simulink model "Dll_Control_AFO_V8_5_R2019b"  (R2019b)
settings: Solver=ode2  StartTime=0.0  StopTime=10  FixedStep=Ts  RelTol=1e-3
InitFcn:
  | modelDir=fileparts(get_param(bdroot,'FileName'));addpath(modelDir);rootDir=fileparts(modelDir);if isfolder(rootDir),addpath(rootDir);end;fmuDir=fullfile(rootDir,'fmu');if isfolder(fmuDir),addpath(fmuDir);end;if evalin('base','exist(''Wf0'',''var'')'),assignin('base','Wfb',evalin('base','Wf0'));end;
values from neighbouring files (symbols this model uses):
  A80 = 0.10573    [RunCtrlSysModelSHT.m]
  b11 = B(1,1)*1    [RunCtrlSysModelSHT.m]
  b21 = B(2,1)*1    [RunCtrlSysModelSHT.m]
  d31 = D(3,1)    [RunCtrlSysModelSHT.m]
  d41 = D(4,1)    [RunCtrlSysModelSHT.m]
  ExternalSecondaryAirEnabled = 0    [RunCtrlSysModelSHT.m]
  InitAir = zeros(50,1)    [RunCtrlSysModelSHT.m]
  Mkg0 = 0    [RunCtrlSysModelSHT.m]
  MkpDirectCommand = Mkp0    (= 999.278795578)    [RunCtrlSysModelSHT.m]
  MkpMax = 1200    [RunCtrlSysModelSHT.m]
  Ng0 = 38000    [RunCtrlSysModelSHT.m]
  NgMax = Ng0*1.05    (= 39900)    [RunCtrlSysModelSHT.m]
  Np0 = 20800    [RunCtrlSysModelSHT.m]
  NpDem = Np0    (= 20800)    [RunCtrlSysModelSHT.m]
  omega_u = 20    [RunCtrlSysModelSHT.m]
  power0 = 2176600    [RunCtrlSysModelSHT.m]
  RotorLoadCfg = struct(      'designNpRpm', Np0,      'designPowerW', power0,      'thetaZeroDeg', 0,      'thetaDesignDeg', 12,      'profileTorqueFraction', 0.15,      'thetaValidRangeDeg', [6, 14])    [RunCtrlSysModelSHT.m]
  RotorLoadInputMode = 'legacyPower'    [RunCtrlSysModelSHT.m]
  T45Max = 1400    [RunCtrlSysModelSHT.m]
  ThetaCommandDeg = RotorLoadCfg.thetaDesignDeg    [RunCtrlSysModelSHT.m]
  Ts = 0.025    [RunCtrlSysModelSHT.m]
  Wf0 = 0.151914044493225    (= 0.151914044493)    [RunCtrlSysModelSHT.m]
  WfMax = Wf0*2    (= 0.303828088986)    [RunCtrlSysModelSHT.m]
  WfMin = Wf0*0.01    (= 0.00151914044493)    [RunCtrlSysModelSHT.m]
  WfRateLim = 1.5    [RunCtrlSysModelSHT.m]
undefined symbols (not defined in the file or in its folder): sigbuilder_block, Wfb
libraries: simulink x10
(part 3 of 4)

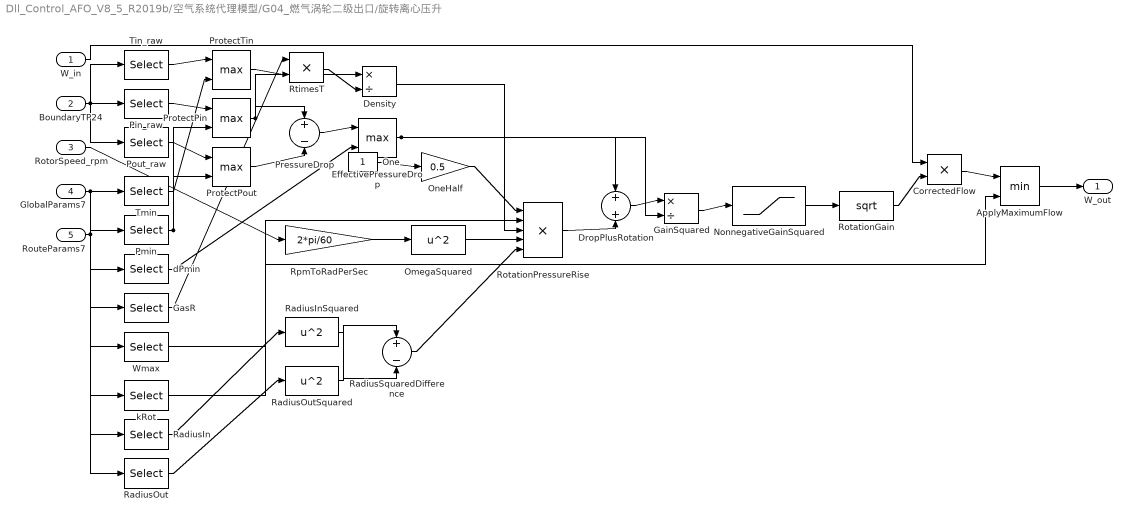
== system Dll_Control_AFO_V8_5_R2019b/空气系统代理模型/G04_燃气涡轮二级出口/旋转离心压升 ==
  W_in : Inport  PortDimensions=1
  BoundaryTP24 : Inport  Port=2  PortDimensions=24
  RotorSpeed_rpm : Inport  Port=3  PortDimensions=1
  GlobalParams7 : Inport  Port=4  PortDimensions=7
  RouteParams7 : Inport  Port=5  PortDimensions=7
  ApplyMaximumFlow : MinMax  Inputs=2
  CorrectedFlow : Product  Inputs=**
  Density : Product  Inputs=*/
  DropPlusRotation : Sum
  EffectivePressureDrop : MinMax  Function=max  Inputs=2
  GainSquared : Product  Inputs=*/
  GasR : Selector  InputPortWidth=7  IndexOptions=Index vector (dialog)  Indices=5  OutputSizes=1
  NonnegativeGainSquared : Saturate  UpperLimit=16  LowerLimit=0
  OmegaSquared : Math  Operator=square  SignedPower=off  SaturateOnIntegerOverflow=on
  One : Constant
  OneHalf : Gain  Gain=0.5
  Pin_raw : Selector  InputPortWidth=24  IndexOptions=Index vector (dialog)  Indices=2*UpstreamBoundary  OutputSizes=1
  Pmin : Selector  InputPortWidth=7  IndexOptions=Index vector (dialog)  Indices=2  OutputSizes=1
  Pout_raw : Selector  InputPortWidth=24  IndexOptions=Index vector (dialog)  Indices=2*DownstreamBoundary  OutputSizes=1
  PressureDrop : Sum  Inputs=+-
  ProtectPin : MinMax  Function=max  Inputs=2
  ProtectPout : MinMax  Function=max  Inputs=2
  ProtectTin : MinMax  Function=max  Inputs=2
  RadiusIn : Selector  InputPortWidth=7  IndexOptions=Index vector (dialog)  Indices=3  OutputSizes=1
  RadiusInSquared : Math  Operator=square  SignedPower=off  SaturateOnIntegerOverflow=on
  RadiusOut : Selector  InputPortWidth=7  IndexOptions=Index vector (dialog)  Indices=4  OutputSizes=1
  RadiusOutSquared : Math  Operator=square  SignedPower=off  SaturateOnIntegerOverflow=on
  RadiusSquaredDifference : Sum  Inputs=+-
  RotationGain : Math  Operator=sqrt  SignedPower=off  SaturateOnIntegerOverflow=on
  RotationPressureRise : Product  Inputs=*****
  RpmToRadPerSec : Gain  Gain=2*pi/60
  RtimesT : Product  Inputs=**
  Tin_raw : Selector  InputPortWidth=24  IndexOptions=Index vector (dialog)  Indices=2*UpstreamBoundary-1  OutputSizes=1
  Tmin : Selector  InputPortWidth=7  IndexOptions=Index vector (dialog)  Indices=1  OutputSizes=1
  Wmax : Selector  InputPortWidth=7  IndexOptions=Index vector (dialog)  Indices=6  OutputSizes=1
  dPmin : Selector  InputPortWidth=7  IndexOptions=Index vector (dialog)  Indices=3  OutputSizes=1
  kRot : Selector  InputPortWidth=7  IndexOptions=Index vector (dialog)  Indices=2  OutputSizes=1
  W_out : Outport
  wires:
  ApplyMaximumFlow/1 -> W_out/1
  Wmax/1 -> ApplyMaximumFlow/2
  CorrectedFlow/1 -> ApplyMaximumFlow/1
  RotationGain/1 -> CorrectedFlow/2
  W_in/1 -> CorrectedFlow/1
  NonnegativeGainSquared/1 -> RotationGain/1
  GainSquared/1 -> NonnegativeGainSquared/1
  DropPlusRotation/1 -> GainSquared/1
  RotationPressureRise/1 -> DropPlusRotation/2
  EffectivePressureDrop/1 -> GainSquared/2, DropPlusRotation/1
  dPmin/1 -> EffectivePressureDrop/2
  PressureDrop/1 -> EffectivePressureDrop/1
  ProtectPout/1 -> PressureDrop/2
  RadiusSquaredDifference/1 -> RotationPressureRise/5
  OmegaSquared/1 -> RotationPressureRise/4
  Density/1 -> RotationPressureRise/3
  kRot/1 -> RotationPressureRise/2
  OneHalf/1 -> RotationPressureRise/1
  One/1 -> OneHalf/1
  RadiusInSquared/1 -> RadiusSquaredDifference/2
  RadiusOutSquared/1 -> RadiusSquaredDifference/1
  RadiusOut/1 -> RadiusOutSquared/1
  RadiusIn/1 -> RadiusInSquared/1
  RpmToRadPerSec/1 -> OmegaSquared/1
  RotorSpeed_rpm/1 -> RpmToRadPerSec/1
  RtimesT/1 -> Density/2
  ProtectPin/1 -> PressureDrop/1, Density/1
  ProtectTin/1 -> RtimesT/2
  GasR/1 -> RtimesT/1
  Pout_raw/1 -> ProtectPout/1
  Pmin/1 -> ProtectPout/2, ProtectPin/2
  Pin_raw/1 -> ProtectPin/1
  Tmin/1 -> ProtectTin/2
  Tin_raw/1 -> ProtectTin/1
  RouteParams7/1 -> RadiusOut/1, RadiusIn/1, kRot/1
  GlobalParams7/1 -> Wmax/1, GasR/1, dPmin/1, Pmin/1, Tmin/1
  BoundaryTP24/1 -> Pout_raw/1, Pin_raw/1, Tin_raw/1

== system Dll_Control_AFO_V8_5_R2019b/空气系统代理模型/G04_燃气涡轮二级出口/流路可调参数 ==
  Mux_RouteParams7 : Mux  Inputs=7
  kRot : Constant  Value=0.5
  内半径_m : Constant  Value=0.074499999999999997
  初值流量_kgps : Constant  Value=0.099328741948656193
  外半径_m : Constant  Value=0.078
  时间常数_s : Constant  Value=0
  等效面积缩放 : Constant  Value=0.9867972125855029
  篦齿修正系数 : Constant
  RouteParams7 : Outport
  wires:
  等效面积缩放/1 -> Mux_RouteParams7/1
  kRot/1 -> Mux_RouteParams7/2
  内半径_m/1 -> Mux_RouteParams7/3
  外半径_m/1 -> Mux_RouteParams7/4
  时间常数_s/1 -> Mux_RouteParams7/5
  初值流量_kgps/1 -> Mux_RouteParams7/6
  篦齿修正系数/1 -> Mux_RouteParams7/7
  Mux_RouteParams7/1 -> RouteParams7/1

== system Dll_Control_AFO_V8_5_R2019b/空气系统代理模型/G04_燃气涡轮二级出口/辨识等效面积 ==
  BoundaryTP24 : Inport  PortDimensions=24
  IdentifiedAreaLaw : MATLAB Function  TreatAsAtomicUnit=on
  EffectiveArea_m2 : Outport
  wires:
  BoundaryTP24/1 -> IdentifiedAreaLaw/1(boundaryTP24)
  IdentifiedAreaLaw/1(area) -> EffectiveArea_m2/1

== system Dll_Control_AFO_V8_5_R2019b/空气系统代理模型/G05_动力涡轮一级叶根进口/可压缩节流孔口 ==
  BoundaryTP24 : Inport  PortDimensions=24
  EffectiveArea_m2 : Inport  Port=2  PortDimensions=1
  GlobalParams7 : Inport  Port=3  PortDimensions=7
  ApplyMaximumFlow : MinMax  Inputs=2
  BoundRatio : Saturate  UpperLimit=1  LowerLimit=1e-6
  CriticalEnabled : Selector  InputPortWidth=7  IndexOptions=Index vector (dialog)  Indices=7  OutputSizes=1
  CriticalRatio : Fcn  Expr=(2/(u+1))^(u/(u-1))
  EnableForwardFlow : Switch  Criteria=u2 ~= 0
  ForwardFlow : RelationalOperator  Operator=>  OutDataTypeStr=boolean  RndMeth=Simplest
  Gamma : Selector  InputPortWidth=7  IndexOptions=Index vector (dialog)  Indices=4  OutputSizes=1
  GasR : Selector  InputPortWidth=7  IndexOptions=Index vector (dialog)  Indices=5  OutputSizes=1
  IsChoked : RelationalOperator  Operator=<=  OutDataTypeStr=boolean  RndMeth=Simplest
  MassFlowRaw : Product  Inputs=***/
  MuxGammaRatio : Mux  Inputs=2
  PhiChoked : Fcn  Expr=sqrt(u)*(2/(u+1))^((u+1)/(2*(u-1)))
  PhiSubcritical : Fcn  Expr=sqrt(2*u(1)/(u(1)-1)*(u(2)^(2/u(1))-u(2)^((u(1)+1)/u(1))))
  Pin_raw : Selector  InputPortWidth=24  IndexOptions=Index vector (dialog)  Indices=2*UpstreamBoundary  OutputSizes=1
  Pmin : Selector  InputPortWidth=7  IndexOptions=Index vector (dialog)  Indices=2  OutputSizes=1
  PoutPlusMinimumDrop : Sum
  Pout_raw : Selector  InputPortWidth=24  IndexOptions=Index vector (dialog)  Indices=2*DownstreamBoundary  OutputSizes=1
  PressureRatio : Product  Inputs=*/
  ProtectPin : MinMax  Function=max  Inputs=2
  ProtectPout : MinMax  Function=max  Inputs=2
  ProtectTin : MinMax  Function=max  Inputs=2
  RT : Product  Inputs=**
  SelectPhi : Switch  Criteria=u2 ~= 0
  SqrtRT : Math  Operator=sqrt  SignedPower=off  SaturateOnIntegerOverflow=on
  Tin_raw : Selector  InputPortWidth=24  IndexOptions=Index vector (dialog)  Indices=2*UpstreamBoundary-1  OutputSizes=1
  Tmin : Selector  InputPortWidth=7  IndexOptions=Index vector (dialog)  Indices=1  OutputSizes=1
  UseChokedBranch : Logic  AllPortsSameDT=off  OutDataTypeStr=boolean
  Wmax : Selector  InputPortWidth=7  IndexOptions=Index vector (dialog)  Indices=6  OutputSizes=1
  ZeroFlow : Constant  Value=0
  dPmin : Selector  InputPortWidth=7  IndexOptions=Index vector (dialog)  Indices=3  OutputSizes=1
  W_kgps : Outport
  wires:
  ApplyMaximumFlow/1 -> W_kgps/1
  Wmax/1 -> ApplyMaximumFlow/2
  EnableForwardFlow/1 -> ApplyMaximumFlow/1
  ZeroFlow/1 -> EnableForwardFlow/3
  ForwardFlow/1 -> EnableForwardFlow/2
  MassFlowRaw/1 -> EnableForwardFlow/1
  SqrtRT/1 -> MassFlowRaw/4
  EffectiveArea_m2/1 -> MassFlowRaw/3
  SelectPhi/1 -> MassFlowRaw/2
  RT/1 -> SqrtRT/1
  ProtectTin/1 -> RT/2
  GasR/1 -> RT/1
  PhiSubcritical/1 -> SelectPhi/3
  UseChokedBranch/1 -> SelectPhi/2
  PhiChoked/1 -> SelectPhi/1
  CriticalEnabled/1 -> UseChokedBranch/2
  IsChoked/1 -> UseChokedBranch/1
  CriticalRatio/1 -> IsChoked/2
  MuxGammaRatio/1 -> PhiSubcritical/1
  BoundRatio/1 -> IsChoked/1, MuxGammaRatio/2
  Gamma/1 -> MuxGammaRatio/1, PhiChoked/1, CriticalRatio/1
  PressureRatio/1 -> BoundRatio/1
  PoutPlusMinimumDrop/1 -> ForwardFlow/2
  ProtectPin/1 -> MassFlowRaw/1, PressureRatio/2, ForwardFlow/1
  dPmin/1 -> PoutPlusMinimumDrop/2
  ProtectPout/1 -> PressureRatio/1, PoutPlusMinimumDrop/1
  Pout_raw/1 -> ProtectPout/1
  Pmin/1 -> ProtectPout/2, ProtectPin/2
  Pin_raw/1 -> ProtectPin/1
  Tmin/1 -> ProtectTin/2
  Tin_raw/1 -> ProtectTin/1
  GlobalParams7/1 -> CriticalEnabled/1, Wmax/1, GasR/1, Gamma/1, dPmin/1, Pmin/1, Tmin/1
  BoundaryTP24/1 -> Pout_raw/1, Pin_raw/1, Tin_raw/1

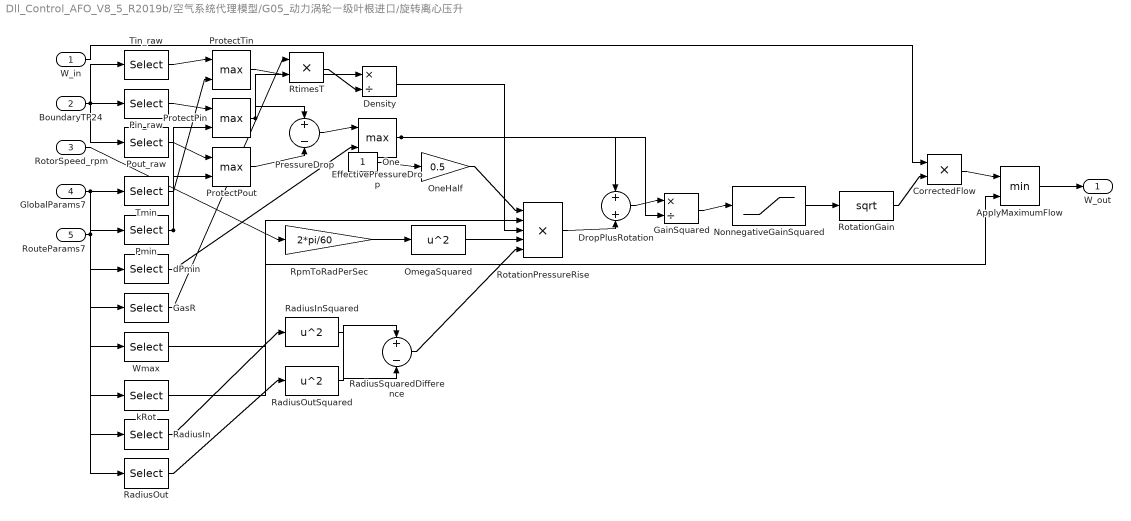
== system Dll_Control_AFO_V8_5_R2019b/空气系统代理模型/G05_动力涡轮一级叶根进口/旋转离心压升 ==
  W_in : Inport  PortDimensions=1
  BoundaryTP24 : Inport  Port=2  PortDimensions=24
  RotorSpeed_rpm : Inport  Port=3  PortDimensions=1
  GlobalParams7 : Inport  Port=4  PortDimensions=7
  RouteParams7 : Inport  Port=5  PortDimensions=7
  ApplyMaximumFlow : MinMax  Inputs=2
  CorrectedFlow : Product  Inputs=**
  Density : Product  Inputs=*/
  DropPlusRotation : Sum
  EffectivePressureDrop : MinMax  Function=max  Inputs=2
  GainSquared : Product  Inputs=*/
  GasR : Selector  InputPortWidth=7  IndexOptions=Index vector (dialog)  Indices=5  OutputSizes=1
  NonnegativeGainSquared : Saturate  UpperLimit=16  LowerLimit=0
  OmegaSquared : Math  Operator=square  SignedPower=off  SaturateOnIntegerOverflow=on
  One : Constant
  OneHalf : Gain  Gain=0.5
  Pin_raw : Selector  InputPortWidth=24  IndexOptions=Index vector (dialog)  Indices=2*UpstreamBoundary  OutputSizes=1
  Pmin : Selector  InputPortWidth=7  IndexOptions=Index vector (dialog)  Indices=2  OutputSizes=1
  Pout_raw : Selector  InputPortWidth=24  IndexOptions=Index vector (dialog)  Indices=2*DownstreamBoundary  OutputSizes=1
  PressureDrop : Sum  Inputs=+-
  ProtectPin : MinMax  Function=max  Inputs=2
  ProtectPout : MinMax  Function=max  Inputs=2
  ProtectTin : MinMax  Function=max  Inputs=2
  RadiusIn : Selector  InputPortWidth=7  IndexOptions=Index vector (dialog)  Indices=3  OutputSizes=1
  RadiusInSquared : Math  Operator=square  SignedPower=off  SaturateOnIntegerOverflow=on
  RadiusOut : Selector  InputPortWidth=7  IndexOptions=Index vector (dialog)  Indices=4  OutputSizes=1
  RadiusOutSquared : Math  Operator=square  SignedPower=off  SaturateOnIntegerOverflow=on
  RadiusSquaredDifference : Sum  Inputs=+-
  RotationGain : Math  Operator=sqrt  SignedPower=off  SaturateOnIntegerOverflow=on
  RotationPressureRise : Product  Inputs=*****
  RpmToRadPerSec : Gain  Gain=2*pi/60
  RtimesT : Product  Inputs=**
  Tin_raw : Selector  InputPortWidth=24  IndexOptions=Index vector (dialog)  Indices=2*UpstreamBoundary-1  OutputSizes=1
  Tmin : Selector  InputPortWidth=7  IndexOptions=Index vector (dialog)  Indices=1  OutputSizes=1
  Wmax : Selector  InputPortWidth=7  IndexOptions=Index vector (dialog)  Indices=6  OutputSizes=1
  dPmin : Selector  InputPortWidth=7  IndexOptions=Index vector (dialog)  Indices=3  OutputSizes=1
  kRot : Selector  InputPortWidth=7  IndexOptions=Index vector (dialog)  Indices=2  OutputSizes=1
  W_out : Outport
  wires:
  ApplyMaximumFlow/1 -> W_out/1
  Wmax/1 -> ApplyMaximumFlow/2
  CorrectedFlow/1 -> ApplyMaximumFlow/1
  RotationGain/1 -> CorrectedFlow/2
  W_in/1 -> CorrectedFlow/1
  NonnegativeGainSquared/1 -> RotationGain/1
  GainSquared/1 -> NonnegativeGainSquared/1
  DropPlusRotation/1 -> GainSquared/1
  RotationPressureRise/1 -> DropPlusRotation/2
  EffectivePressureDrop/1 -> GainSquared/2, DropPlusRotation/1
  dPmin/1 -> EffectivePressureDrop/2
  PressureDrop/1 -> EffectivePressureDrop/1
  ProtectPout/1 -> PressureDrop/2
  RadiusSquaredDifference/1 -> RotationPressureRise/5
  OmegaSquared/1 -> RotationPressureRise/4
  Density/1 -> RotationPressureRise/3
  kRot/1 -> RotationPressureRise/2
  OneHalf/1 -> RotationPressureRise/1
  One/1 -> OneHalf/1
  RadiusInSquared/1 -> RadiusSquaredDifference/2
  RadiusOutSquared/1 -> RadiusSquaredDifference/1
  RadiusOut/1 -> RadiusOutSquared/1
  RadiusIn/1 -> RadiusInSquared/1
  RpmToRadPerSec/1 -> OmegaSquared/1
  RotorSpeed_rpm/1 -> RpmToRadPerSec/1
  RtimesT/1 -> Density/2
  ProtectPin/1 -> PressureDrop/1, Density/1
  ProtectTin/1 -> RtimesT/2
  GasR/1 -> RtimesT/1
  Pout_raw/1 -> ProtectPout/1
  Pmin/1 -> ProtectPout/2, ProtectPin/2
  Pin_raw/1 -> ProtectPin/1
  Tmin/1 -> ProtectTin/2
  Tin_raw/1 -> ProtectTin/1
  RouteParams7/1 -> RadiusOut/1, RadiusIn/1, kRot/1
  GlobalParams7/1 -> Wmax/1, GasR/1, dPmin/1, Pmin/1, Tmin/1
  BoundaryTP24/1 -> Pout_raw/1, Pin_raw/1, Tin_raw/1

== system Dll_Control_AFO_V8_5_R2019b/空气系统代理模型/G05_动力涡轮一级叶根进口/流路可调参数 ==
  Mux_RouteParams7 : Mux  Inputs=7
  kRot : Constant  Value=0.5
  内半径_m : Constant  Value=0.053999999999999999
  初值流量_kgps : Constant  Value=0.038254988453198698
  外半径_m : Constant  Value=0.059499999999999997
  时间常数_s : Constant  Value=0
  等效面积缩放 : Constant  Value=0.989491921844591
  篦齿修正系数 : Constant
  RouteParams7 : Outport
  wires:
  等效面积缩放/1 -> Mux_RouteParams7/1
  kRot/1 -> Mux_RouteParams7/2
  内半径_m/1 -> Mux_RouteParams7/3
  外半径_m/1 -> Mux_RouteParams7/4
  时间常数_s/1 -> Mux_RouteParams7/5
  初值流量_kgps/1 -> Mux_RouteParams7/6
  篦齿修正系数/1 -> Mux_RouteParams7/7
  Mux_RouteParams7/1 -> RouteParams7/1

== system Dll_Control_AFO_V8_5_R2019b/空气系统代理模型/G05_动力涡轮一级叶根进口/盘腔热动态 ==
  W_in : Inport  PortDimensions=1
  RouteParams7 : Inport  Port=2  PortDimensions=7
  Alpha : Fcn  Expr=exp(-SampleTime_s/u)
  DynamicOrBypass : Switch  Criteria=u2 ~= 0
  One : Constant
  OneMinusAlpha : Sum  Inputs=+-
  ProtectTau : Saturate  UpperLimit=inf  LowerLimit=1e-9
  State : UnitDelay  InitialCondition=InitialFlowValue  SampleTime=SampleTime_s  HasFrameUpgradeWarning=on
  Tau_s : Selector  InputPortWidth=7  IndexOptions=Index vector (dialog)  Indices=5  OutputSizes=1
  Update : Sum
  UseBypass : simulink/Logic and Bit Operations/Compare To Constant  relop=<=  const=1e-12  OutDataTypeStr=boolean
  WeightedInput : Product  Inputs=**
  WeightedState : Product  Inputs=**
  W_out : Outport
  wires:
  DynamicOrBypass/1 -> W_out/1
  UseBypass/1 -> DynamicOrBypass/2
  Update/1 -> DynamicOrBypass/3, State/1
  WeightedState/1 -> Update/2
  WeightedInput/1 -> Update/1
  State/1 -> WeightedState/1
  OneMinusAlpha/1 -> WeightedInput/2
  W_in/1 -> DynamicOrBypass/1, WeightedInput/1
  Alpha/1 -> WeightedState/2, OneMinusAlpha/2
  One/1 -> OneMinusAlpha/1
  ProtectTau/1 -> Alpha/1
  Tau_s/1 -> UseBypass/1, ProtectTau/1
  RouteParams7/1 -> Tau_s/1

== system Dll_Control_AFO_V8_5_R2019b/空气系统代理模型/G05_动力涡轮一级叶根进口/辨识等效面积 ==
  BoundaryTP24 : Inport  PortDimensions=24
  IdentifiedAreaLaw : MATLAB Function  TreatAsAtomicUnit=on
  EffectiveArea_m2 : Outport
  wires:
  BoundaryTP24/1 -> IdentifiedAreaLaw/1(boundaryTP24)
  IdentifiedAreaLaw/1(area) -> EffectiveArea_m2/1

== system Dll_Control_AFO_V8_5_R2019b/空气系统代理模型/G06_动力涡轮一级叶根出口/可压缩节流孔口 ==
  BoundaryTP24 : Inport  PortDimensions=24
  EffectiveArea_m2 : Inport  Port=2  PortDimensions=1
  GlobalParams7 : Inport  Port=3  PortDimensions=7
  ApplyMaximumFlow : MinMax  Inputs=2
  BoundRatio : Saturate  UpperLimit=1  LowerLimit=1e-6
  CriticalEnabled : Selector  InputPortWidth=7  IndexOptions=Index vector (dialog)  Indices=7  OutputSizes=1
  CriticalRatio : Fcn  Expr=(2/(u+1))^(u/(u-1))
  EnableForwardFlow : Switch  Criteria=u2 ~= 0
  ForwardFlow : RelationalOperator  Operator=>  OutDataTypeStr=boolean  RndMeth=Simplest
  Gamma : Selector  InputPortWidth=7  IndexOptions=Index vector (dialog)  Indices=4  OutputSizes=1
  GasR : Selector  InputPortWidth=7  IndexOptions=Index vector (dialog)  Indices=5  OutputSizes=1
  IsChoked : RelationalOperator  Operator=<=  OutDataTypeStr=boolean  RndMeth=Simplest
  MassFlowRaw : Product  Inputs=***/
  MuxGammaRatio : Mux  Inputs=2
  PhiChoked : Fcn  Expr=sqrt(u)*(2/(u+1))^((u+1)/(2*(u-1)))
  PhiSubcritical : Fcn  Expr=sqrt(2*u(1)/(u(1)-1)*(u(2)^(2/u(1))-u(2)^((u(1)+1)/u(1))))
  Pin_raw : Selector  InputPortWidth=24  IndexOptions=Index vector (dialog)  Indices=2*UpstreamBoundary  OutputSizes=1
  Pmin : Selector  InputPortWidth=7  IndexOptions=Index vector (dialog)  Indices=2  OutputSizes=1
  PoutPlusMinimumDrop : Sum
  Pout_raw : Selector  InputPortWidth=24  IndexOptions=Index vector (dialog)  Indices=2*DownstreamBoundary  OutputSizes=1
  PressureRatio : Product  Inputs=*/
  ProtectPin : MinMax  Function=max  Inputs=2
  ProtectPout : MinMax  Function=max  Inputs=2
  ProtectTin : MinMax  Function=max  Inputs=2
  RT : Product  Inputs=**
  SelectPhi : Switch  Criteria=u2 ~= 0
  SqrtRT : Math  Operator=sqrt  SignedPower=off  SaturateOnIntegerOverflow=on
  Tin_raw : Selector  InputPortWidth=24  IndexOptions=Index vector (dialog)  Indices=2*UpstreamBoundary-1  OutputSizes=1
  Tmin : Selector  InputPortWidth=7  IndexOptions=Index vector (dialog)  Indices=1  OutputSizes=1
  UseChokedBranch : Logic  AllPortsSameDT=off  OutDataTypeStr=boolean
  Wmax : Selector  InputPortWidth=7  IndexOptions=Index vector (dialog)  Indices=6  OutputSizes=1
  ZeroFlow : Constant  Value=0
  dPmin : Selector  InputPortWidth=7  IndexOptions=Index vector (dialog)  Indices=3  OutputSizes=1
  W_kgps : Outport
  wires:
  ApplyMaximumFlow/1 -> W_kgps/1
  Wmax/1 -> ApplyMaximumFlow/2
  EnableForwardFlow/1 -> ApplyMaximumFlow/1
  ZeroFlow/1 -> EnableForwardFlow/3
  ForwardFlow/1 -> EnableForwardFlow/2
  MassFlowRaw/1 -> EnableForwardFlow/1
  SqrtRT/1 -> MassFlowRaw/4
  EffectiveArea_m2/1 -> MassFlowRaw/3
  SelectPhi/1 -> MassFlowRaw/2
  RT/1 -> SqrtRT/1
  ProtectTin/1 -> RT/2
  GasR/1 -> RT/1
  PhiSubcritical/1 -> SelectPhi/3
  UseChokedBranch/1 -> SelectPhi/2
  PhiChoked/1 -> SelectPhi/1
  CriticalEnabled/1 -> UseChokedBranch/2
  IsChoked/1 -> UseChokedBranch/1
  CriticalRatio/1 -> IsChoked/2
  MuxGammaRatio/1 -> PhiSubcritical/1
  BoundRatio/1 -> IsChoked/1, MuxGammaRatio/2
  Gamma/1 -> MuxGammaRatio/1, PhiChoked/1, CriticalRatio/1
  PressureRatio/1 -> BoundRatio/1
  PoutPlusMinimumDrop/1 -> ForwardFlow/2
  ProtectPin/1 -> MassFlowRaw/1, PressureRatio/2, ForwardFlow/1
  dPmin/1 -> PoutPlusMinimumDrop/2
  ProtectPout/1 -> PressureRatio/1, PoutPlusMinimumDrop/1
  Pout_raw/1 -> ProtectPout/1
  Pmin/1 -> ProtectPout/2, ProtectPin/2
  Pin_raw/1 -> ProtectPin/1
  Tmin/1 -> ProtectTin/2
  Tin_raw/1 -> ProtectTin/1
  GlobalParams7/1 -> CriticalEnabled/1, Wmax/1, GasR/1, Gamma/1, dPmin/1, Pmin/1, Tmin/1
  BoundaryTP24/1 -> Pout_raw/1, Pin_raw/1, Tin_raw/1

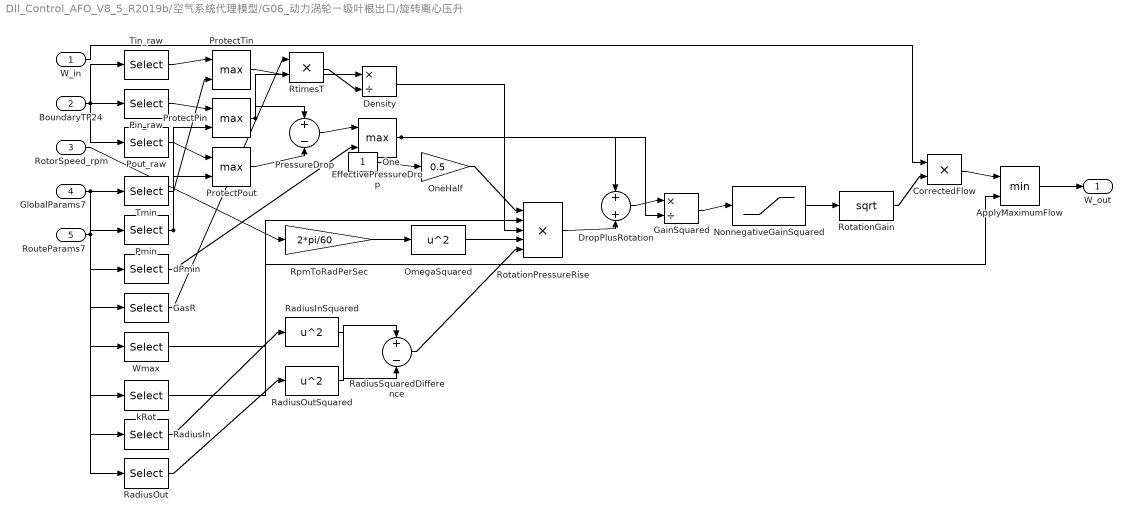
== system Dll_Control_AFO_V8_5_R2019b/空气系统代理模型/G06_动力涡轮一级叶根出口/旋转离心压升 ==
  W_in : Inport  PortDimensions=1
  BoundaryTP24 : Inport  Port=2  PortDimensions=24
  RotorSpeed_rpm : Inport  Port=3  PortDimensions=1
  GlobalParams7 : Inport  Port=4  PortDimensions=7
  RouteParams7 : Inport  Port=5  PortDimensions=7
  ApplyMaximumFlow : MinMax  Inputs=2
  CorrectedFlow : Product  Inputs=**
  Density : Product  Inputs=*/
  DropPlusRotation : Sum
  EffectivePressureDrop : MinMax  Function=max  Inputs=2
  GainSquared : Product  Inputs=*/
  GasR : Selector  InputPortWidth=7  IndexOptions=Index vector (dialog)  Indices=5  OutputSizes=1
  NonnegativeGainSquared : Saturate  UpperLimit=16  LowerLimit=0
  OmegaSquared : Math  Operator=square  SignedPower=off  SaturateOnIntegerOverflow=on
  One : Constant
  OneHalf : Gain  Gain=0.5
  Pin_raw : Selector  InputPortWidth=24  IndexOptions=Index vector (dialog)  Indices=2*UpstreamBoundary  OutputSizes=1
  Pmin : Selector  InputPortWidth=7  IndexOptions=Index vector (dialog)  Indices=2  OutputSizes=1
  Pout_raw : Selector  InputPortWidth=24  IndexOptions=Index vector (dialog)  Indices=2*DownstreamBoundary  OutputSizes=1
  PressureDrop : Sum  Inputs=+-
  ProtectPin : MinMax  Function=max  Inputs=2
  ProtectPout : MinMax  Function=max  Inputs=2
  ProtectTin : MinMax  Function=max  Inputs=2
  RadiusIn : Selector  InputPortWidth=7  IndexOptions=Index vector (dialog)  Indices=3  OutputSizes=1
  RadiusInSquared : Math  Operator=square  SignedPower=off  SaturateOnIntegerOverflow=on
  RadiusOut : Selector  InputPortWidth=7  IndexOptions=Index vector (dialog)  Indices=4  OutputSizes=1
  RadiusOutSquared : Math  Operator=square  SignedPower=off  SaturateOnIntegerOverflow=on
  RadiusSquaredDifference : Sum  Inputs=+-
  RotationGain : Math  Operator=sqrt  SignedPower=off  SaturateOnIntegerOverflow=on
  RotationPressureRise : Product  Inputs=*****
  RpmToRadPerSec : Gain  Gain=2*pi/60
  RtimesT : Product  Inputs=**
  Tin_raw : Selector  InputPortWidth=24  IndexOptions=Index vector (dialog)  Indices=2*UpstreamBoundary-1  OutputSizes=1
  Tmin : Selector  InputPortWidth=7  IndexOptions=Index vector (dialog)  Indices=1  OutputSizes=1
  Wmax : Selector  InputPortWidth=7  IndexOptions=Index vector (dialog)  Indices=6  OutputSizes=1
  dPmin : Selector  InputPortWidth=7  IndexOptions=Index vector (dialog)  Indices=3  OutputSizes=1
  kRot : Selector  InputPortWidth=7  IndexOptions=Index vector (dialog)  Indices=2  OutputSizes=1
  W_out : Outport
  wires:
  ApplyMaximumFlow/1 -> W_out/1
  Wmax/1 -> ApplyMaximumFlow/2
  CorrectedFlow/1 -> ApplyMaximumFlow/1
  RotationGain/1 -> CorrectedFlow/2
  W_in/1 -> CorrectedFlow/1
  NonnegativeGainSquared/1 -> RotationGain/1
  GainSquared/1 -> NonnegativeGainSquared/1
  DropPlusRotation/1 -> GainSquared/1
  RotationPressureRise/1 -> DropPlusRotation/2
  EffectivePressureDrop/1 -> GainSquared/2, DropPlusRotation/1
  dPmin/1 -> EffectivePressureDrop/2
  PressureDrop/1 -> EffectivePressureDrop/1
  ProtectPout/1 -> PressureDrop/2
  RadiusSquaredDifference/1 -> RotationPressureRise/5
  OmegaSquared/1 -> RotationPressureRise/4
  Density/1 -> RotationPressureRise/3
  kRot/1 -> RotationPressureRise/2
  OneHalf/1 -> RotationPressureRise/1
  One/1 -> OneHalf/1
  RadiusInSquared/1 -> RadiusSquaredDifference/2
  RadiusOutSquared/1 -> RadiusSquaredDifference/1
  RadiusOut/1 -> RadiusOutSquared/1
  RadiusIn/1 -> RadiusInSquared/1
  RpmToRadPerSec/1 -> OmegaSquared/1
  RotorSpeed_rpm/1 -> RpmToRadPerSec/1
  RtimesT/1 -> Density/2
  ProtectPin/1 -> PressureDrop/1, Density/1
  ProtectTin/1 -> RtimesT/2
  GasR/1 -> RtimesT/1
  Pout_raw/1 -> ProtectPout/1
  Pmin/1 -> ProtectPout/2, ProtectPin/2
  Pin_raw/1 -> ProtectPin/1
  Tmin/1 -> ProtectTin/2
  Tin_raw/1 -> ProtectTin/1
  RouteParams7/1 -> RadiusOut/1, RadiusIn/1, kRot/1
  GlobalParams7/1 -> Wmax/1, GasR/1, dPmin/1, Pmin/1, Tmin/1
  BoundaryTP24/1 -> Pout_raw/1, Pin_raw/1, Tin_raw/1

== system Dll_Control_AFO_V8_5_R2019b/空气系统代理模型/G06_动力涡轮一级叶根出口/流路可调参数 ==
  Mux_RouteParams7 : Mux  Inputs=7
  kRot : Constant  Value=0.5
  内半径_m : Constant  Value=0.059499999999999997
  初值流量_kgps : Constant  Value=0.0308724468218796
  外半径_m : Constant  Value=0.074499999999999997
  时间常数_s : Constant  Value=0
  等效面积缩放 : Constant  Value=0.989425808658701
  篦齿修正系数 : Constant
  RouteParams7 : Outport
  wires:
  等效面积缩放/1 -> Mux_RouteParams7/1
  kRot/1 -> Mux_RouteParams7/2
  内半径_m/1 -> Mux_RouteParams7/3
  外半径_m/1 -> Mux_RouteParams7/4
  时间常数_s/1 -> Mux_RouteParams7/5
  初值流量_kgps/1 -> Mux_RouteParams7/6
  篦齿修正系数/1 -> Mux_RouteParams7/7
  Mux_RouteParams7/1 -> RouteParams7/1

== system Dll_Control_AFO_V8_5_R2019b/空气系统代理模型/G06_动力涡轮一级叶根出口/盘腔热动态 ==
  W_in : Inport  PortDimensions=1
  RouteParams7 : Inport  Port=2  PortDimensions=7
  Alpha : Fcn  Expr=exp(-SampleTime_s/u)
  DynamicOrBypass : Switch  Criteria=u2 ~= 0
  One : Constant
  OneMinusAlpha : Sum  Inputs=+-
  ProtectTau : Saturate  UpperLimit=inf  LowerLimit=1e-9
  State : UnitDelay  InitialCondition=InitialFlowValue  SampleTime=SampleTime_s  HasFrameUpgradeWarning=on
  Tau_s : Selector  InputPortWidth=7  IndexOptions=Index vector (dialog)  Indices=5  OutputSizes=1
  Update : Sum
  UseBypass : simulink/Logic and Bit Operations/Compare To Constant  relop=<=  const=1e-12  OutDataTypeStr=boolean
  WeightedInput : Product  Inputs=**
  WeightedState : Product  Inputs=**
  W_out : Outport
  wires:
  DynamicOrBypass/1 -> W_out/1
  UseBypass/1 -> DynamicOrBypass/2
  Update/1 -> DynamicOrBypass/3, State/1
  WeightedState/1 -> Update/2
  WeightedInput/1 -> Update/1
  State/1 -> WeightedState/1
  OneMinusAlpha/1 -> WeightedInput/2
  W_in/1 -> DynamicOrBypass/1, WeightedInput/1
  Alpha/1 -> WeightedState/2, OneMinusAlpha/2
  One/1 -> OneMinusAlpha/1
  ProtectTau/1 -> Alpha/1
  Tau_s/1 -> UseBypass/1, ProtectTau/1
  RouteParams7/1 -> Tau_s/1

== system Dll_Control_AFO_V8_5_R2019b/空气系统代理模型/G06_动力涡轮一级叶根出口/辨识等效面积 ==
  BoundaryTP24 : Inport  PortDimensions=24
  IdentifiedAreaLaw : MATLAB Function  TreatAsAtomicUnit=on
  EffectiveArea_m2 : Outport
  wires:
  BoundaryTP24/1 -> IdentifiedAreaLaw/1(boundaryTP24)
  IdentifiedAreaLaw/1(area) -> EffectiveArea_m2/1

== system Dll_Control_AFO_V8_5_R2019b/空气系统代理模型/G07_动力涡轮二级叶尖进口/可压缩节流孔口 ==
  BoundaryTP24 : Inport  PortDimensions=24
  EffectiveArea_m2 : Inport  Port=2  PortDimensions=1
  GlobalParams7 : Inport  Port=3  PortDimensions=7
  ApplyMaximumFlow : MinMax  Inputs=2
  BoundRatio : Saturate  UpperLimit=1  LowerLimit=1e-6
  CriticalEnabled : Selector  InputPortWidth=7  IndexOptions=Index vector (dialog)  Indices=7  OutputSizes=1
  CriticalRatio : Fcn  Expr=(2/(u+1))^(u/(u-1))
  EnableForwardFlow : Switch  Criteria=u2 ~= 0
  ForwardFlow : RelationalOperator  Operator=>  OutDataTypeStr=boolean  RndMeth=Simplest
  Gamma : Selector  InputPortWidth=7  IndexOptions=Index vector (dialog)  Indices=4  OutputSizes=1
  GasR : Selector  InputPortWidth=7  IndexOptions=Index vector (dialog)  Indices=5  OutputSizes=1
  IsChoked : RelationalOperator  Operator=<=  OutDataTypeStr=boolean  RndMeth=Simplest
  MassFlowRaw : Product  Inputs=***/
  MuxGammaRatio : Mux  Inputs=2
  PhiChoked : Fcn  Expr=sqrt(u)*(2/(u+1))^((u+1)/(2*(u-1)))
  PhiSubcritical : Fcn  Expr=sqrt(2*u(1)/(u(1)-1)*(u(2)^(2/u(1))-u(2)^((u(1)+1)/u(1))))
  Pin_raw : Selector  InputPortWidth=24  IndexOptions=Index vector (dialog)  Indices=2*UpstreamBoundary  OutputSizes=1
  Pmin : Selector  InputPortWidth=7  IndexOptions=Index vector (dialog)  Indices=2  OutputSizes=1
  PoutPlusMinimumDrop : Sum
  Pout_raw : Selector  InputPortWidth=24  IndexOptions=Index vector (dialog)  Indices=2*DownstreamBoundary  OutputSizes=1
  PressureRatio : Product  Inputs=*/
  ProtectPin : MinMax  Function=max  Inputs=2
  ProtectPout : MinMax  Function=max  Inputs=2
  ProtectTin : MinMax  Function=max  Inputs=2
  RT : Product  Inputs=**
  SelectPhi : Switch  Criteria=u2 ~= 0
  SqrtRT : Math  Operator=sqrt  SignedPower=off  SaturateOnIntegerOverflow=on
  Tin_raw : Selector  InputPortWidth=24  IndexOptions=Index vector (dialog)  Indices=2*UpstreamBoundary-1  OutputSizes=1
  Tmin : Selector  InputPortWidth=7  IndexOptions=Index vector (dialog)  Indices=1  OutputSizes=1
  UseChokedBranch : Logic  AllPortsSameDT=off  OutDataTypeStr=boolean
  Wmax : Selector  InputPortWidth=7  IndexOptions=Index vector (dialog)  Indices=6  OutputSizes=1
  ZeroFlow : Constant  Value=0
  dPmin : Selector  InputPortWidth=7  IndexOptions=Index vector (dialog)  Indices=3  OutputSizes=1
  W_kgps : Outport
  wires:
  ApplyMaximumFlow/1 -> W_kgps/1
  Wmax/1 -> ApplyMaximumFlow/2
  EnableForwardFlow/1 -> ApplyMaximumFlow/1
  ZeroFlow/1 -> EnableForwardFlow/3
  ForwardFlow/1 -> EnableForwardFlow/2
  MassFlowRaw/1 -> EnableForwardFlow/1
  SqrtRT/1 -> MassFlowRaw/4
  EffectiveArea_m2/1 -> MassFlowRaw/3
  SelectPhi/1 -> MassFlowRaw/2
  RT/1 -> SqrtRT/1
  ProtectTin/1 -> RT/2
  GasR/1 -> RT/1
  PhiSubcritical/1 -> SelectPhi/3
  UseChokedBranch/1 -> SelectPhi/2
  PhiChoked/1 -> SelectPhi/1
  CriticalEnabled/1 -> UseChokedBranch/2
  IsChoked/1 -> UseChokedBranch/1
  CriticalRatio/1 -> IsChoked/2
  MuxGammaRatio/1 -> PhiSubcritical/1
  BoundRatio/1 -> IsChoked/1, MuxGammaRatio/2
  Gamma/1 -> MuxGammaRatio/1, PhiChoked/1, CriticalRatio/1
  PressureRatio/1 -> BoundRatio/1
  PoutPlusMinimumDrop/1 -> ForwardFlow/2
  ProtectPin/1 -> MassFlowRaw/1, PressureRatio/2, ForwardFlow/1
  dPmin/1 -> PoutPlusMinimumDrop/2
  ProtectPout/1 -> PressureRatio/1, PoutPlusMinimumDrop/1
  Pout_raw/1 -> ProtectPout/1
  Pmin/1 -> ProtectPout/2, ProtectPin/2
  Pin_raw/1 -> ProtectPin/1
  Tmin/1 -> ProtectTin/2
  Tin_raw/1 -> ProtectTin/1
  GlobalParams7/1 -> CriticalEnabled/1, Wmax/1, GasR/1, Gamma/1, dPmin/1, Pmin/1, Tmin/1
  BoundaryTP24/1 -> Pout_raw/1, Pin_raw/1, Tin_raw/1

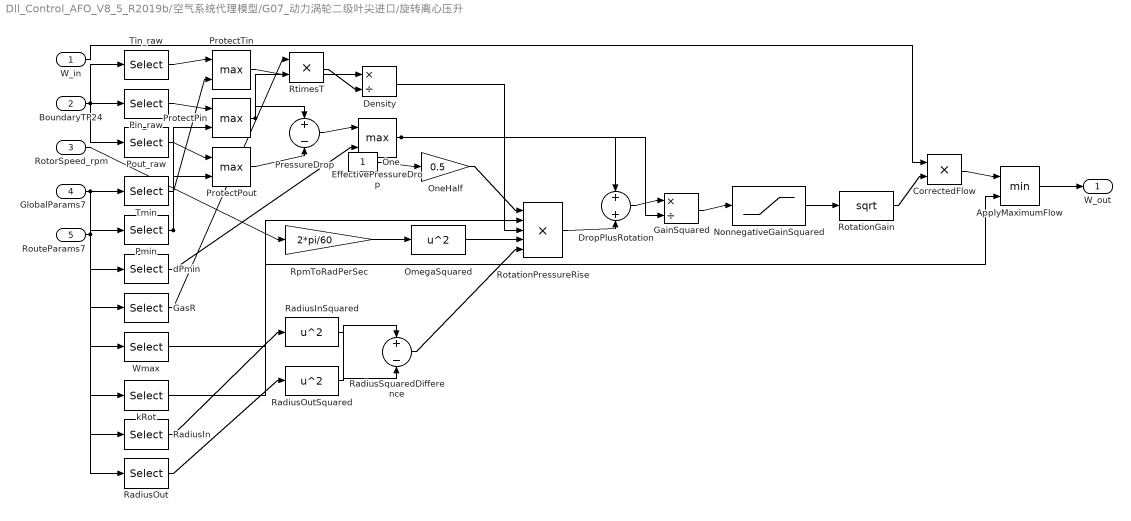
== system Dll_Control_AFO_V8_5_R2019b/空气系统代理模型/G07_动力涡轮二级叶尖进口/旋转离心压升 ==
  W_in : Inport  PortDimensions=1
  BoundaryTP24 : Inport  Port=2  PortDimensions=24
  RotorSpeed_rpm : Inport  Port=3  PortDimensions=1
  GlobalParams7 : Inport  Port=4  PortDimensions=7
  RouteParams7 : Inport  Port=5  PortDimensions=7
  ApplyMaximumFlow : MinMax  Inputs=2
  CorrectedFlow : Product  Inputs=**
  Density : Product  Inputs=*/
  DropPlusRotation : Sum
  EffectivePressureDrop : MinMax  Function=max  Inputs=2
  GainSquared : Product  Inputs=*/
  GasR : Selector  InputPortWidth=7  IndexOptions=Index vector (dialog)  Indices=5  OutputSizes=1
  NonnegativeGainSquared : Saturate  UpperLimit=16  LowerLimit=0
  OmegaSquared : Math  Operator=square  SignedPower=off  SaturateOnIntegerOverflow=on
  One : Constant
  OneHalf : Gain  Gain=0.5
  Pin_raw : Selector  InputPortWidth=24  IndexOptions=Index vector (dialog)  Indices=2*UpstreamBoundary  OutputSizes=1
  Pmin : Selector  InputPortWidth=7  IndexOptions=Index vector (dialog)  Indices=2  OutputSizes=1
  Pout_raw : Selector  InputPortWidth=24  IndexOptions=Index vector (dialog)  Indices=2*DownstreamBoundary  OutputSizes=1
  PressureDrop : Sum  Inputs=+-
  ProtectPin : MinMax  Function=max  Inputs=2
  ProtectPout : MinMax  Function=max  Inputs=2
  ProtectTin : MinMax  Function=max  Inputs=2
  RadiusIn : Selector  InputPortWidth=7  IndexOptions=Index vector (dialog)  Indices=3  OutputSizes=1
  RadiusInSquared : Math  Operator=square  SignedPower=off  SaturateOnIntegerOverflow=on
  RadiusOut : Selector  InputPortWidth=7  IndexOptions=Index vector (dialog)  Indices=4  OutputSizes=1
  RadiusOutSquared : Math  Operator=square  SignedPower=off  SaturateOnIntegerOverflow=on
  RadiusSquaredDifference : Sum  Inputs=+-
  RotationGain : Math  Operator=sqrt  SignedPower=off  SaturateOnIntegerOverflow=on
  RotationPressureRise : Product  Inputs=*****
  RpmToRadPerSec : Gain  Gain=2*pi/60
  RtimesT : Product  Inputs=**
  Tin_raw : Selector  InputPortWidth=24  IndexOptions=Index vector (dialog)  Indices=2*UpstreamBoundary-1  OutputSizes=1
  Tmin : Selector  InputPortWidth=7  IndexOptions=Index vector (dialog)  Indices=1  OutputSizes=1
  Wmax : Selector  InputPortWidth=7  IndexOptions=Index vector (dialog)  Indices=6  OutputSizes=1
  dPmin : Selector  InputPortWidth=7  IndexOptions=Index vector (dialog)  Indices=3  OutputSizes=1
  kRot : Selector  InputPortWidth=7  IndexOptions=Index vector (dialog)  Indices=2  OutputSizes=1
  W_out : Outport
  wires:
  ApplyMaximumFlow/1 -> W_out/1
  Wmax/1 -> ApplyMaximumFlow/2
  CorrectedFlow/1 -> ApplyMaximumFlow/1
  RotationGain/1 -> CorrectedFlow/2
  W_in/1 -> CorrectedFlow/1
  NonnegativeGainSquared/1 -> RotationGain/1
  GainSquared/1 -> NonnegativeGainSquared/1
  DropPlusRotation/1 -> GainSquared/1
  RotationPressureRise/1 -> DropPlusRotation/2
  EffectivePressureDrop/1 -> GainSquared/2, DropPlusRotation/1
  dPmin/1 -> EffectivePressureDrop/2
  PressureDrop/1 -> EffectivePressureDrop/1
  ProtectPout/1 -> PressureDrop/2
  RadiusSquaredDifference/1 -> RotationPressureRise/5
  OmegaSquared/1 -> RotationPressureRise/4
  Density/1 -> RotationPressureRise/3
  kRot/1 -> RotationPressureRise/2
  OneHalf/1 -> RotationPressureRise/1
  One/1 -> OneHalf/1
  RadiusInSquared/1 -> RadiusSquaredDifference/2
  RadiusOutSquared/1 -> RadiusSquaredDifference/1
  RadiusOut/1 -> RadiusOutSquared/1
  RadiusIn/1 -> RadiusInSquared/1
  RpmToRadPerSec/1 -> OmegaSquared/1
  RotorSpeed_rpm/1 -> RpmToRadPerSec/1
  RtimesT/1 -> Density/2
  ProtectPin/1 -> PressureDrop/1, Density/1
  ProtectTin/1 -> RtimesT/2
  GasR/1 -> RtimesT/1
  Pout_raw/1 -> ProtectPout/1
  Pmin/1 -> ProtectPout/2, ProtectPin/2
  Pin_raw/1 -> ProtectPin/1
  Tmin/1 -> ProtectTin/2
  Tin_raw/1 -> ProtectTin/1
  RouteParams7/1 -> RadiusOut/1, RadiusIn/1, kRot/1
  GlobalParams7/1 -> Wmax/1, GasR/1, dPmin/1, Pmin/1, Tmin/1
  BoundaryTP24/1 -> Pout_raw/1, Pin_raw/1, Tin_raw/1

== system Dll_Control_AFO_V8_5_R2019b/空气系统代理模型/G07_动力涡轮二级叶尖进口/流路可调参数 ==
  Mux_RouteParams7 : Mux  Inputs=7
  kRot : Constant  Value=0.5
  内半径_m : Constant  Value=0.074499999999999997
  初值流量_kgps : Constant  Value=0.042952969491310798
  外半径_m : Constant  Value=0.076999999999999999
  时间常数_s : Constant  Value=0
  等效面积缩放 : Constant  Value=1.0010878893618813
  篦齿修正系数 : Constant
  RouteParams7 : Outport
  wires:
  等效面积缩放/1 -> Mux_RouteParams7/1
  kRot/1 -> Mux_RouteParams7/2
  内半径_m/1 -> Mux_RouteParams7/3
  外半径_m/1 -> Mux_RouteParams7/4
  时间常数_s/1 -> Mux_RouteParams7/5
  初值流量_kgps/1 -> Mux_RouteParams7/6
  篦齿修正系数/1 -> Mux_RouteParams7/7
  Mux_RouteParams7/1 -> RouteParams7/1

== system Dll_Control_AFO_V8_5_R2019b/空气系统代理模型/G07_动力涡轮二级叶尖进口/盘腔热动态 ==
  W_in : Inport  PortDimensions=1
  RouteParams7 : Inport  Port=2  PortDimensions=7
  Alpha : Fcn  Expr=exp(-SampleTime_s/u)
  DynamicOrBypass : Switch  Criteria=u2 ~= 0
  One : Constant
  OneMinusAlpha : Sum  Inputs=+-
  ProtectTau : Saturate  UpperLimit=inf  LowerLimit=1e-9
  State : UnitDelay  InitialCondition=InitialFlowValue  SampleTime=SampleTime_s  HasFrameUpgradeWarning=on
  Tau_s : Selector  InputPortWidth=7  IndexOptions=Index vector (dialog)  Indices=5  OutputSizes=1
  Update : Sum
  UseBypass : simulink/Logic and Bit Operations/Compare To Constant  relop=<=  const=1e-12  OutDataTypeStr=boolean
  WeightedInput : Product  Inputs=**
  WeightedState : Product  Inputs=**
  W_out : Outport
  wires:
  DynamicOrBypass/1 -> W_out/1
  UseBypass/1 -> DynamicOrBypass/2
  Update/1 -> DynamicOrBypass/3, State/1
  WeightedState/1 -> Update/2
  WeightedInput/1 -> Update/1
  State/1 -> WeightedState/1
  OneMinusAlpha/1 -> WeightedInput/2
  W_in/1 -> DynamicOrBypass/1, WeightedInput/1
  Alpha/1 -> WeightedState/2, OneMinusAlpha/2
  One/1 -> OneMinusAlpha/1
  ProtectTau/1 -> Alpha/1
  Tau_s/1 -> UseBypass/1, ProtectTau/1
  RouteParams7/1 -> Tau_s/1

== system Dll_Control_AFO_V8_5_R2019b/空气系统代理模型/G07_动力涡轮二级叶尖进口/辨识等效面积 ==
  BoundaryTP24 : Inport  PortDimensions=24
  IdentifiedAreaLaw : MATLAB Function  TreatAsAtomicUnit=on
  EffectiveArea_m2 : Outport
  wires:
  BoundaryTP24/1 -> IdentifiedAreaLaw/1(boundaryTP24)
  IdentifiedAreaLaw/1(area) -> EffectiveArea_m2/1

== system Dll_Control_AFO_V8_5_R2019b/空气系统代理模型/G08_动力涡轮二级叶尖出口/可压缩节流孔口 ==
  BoundaryTP24 : Inport  PortDimensions=24
  EffectiveArea_m2 : Inport  Port=2  PortDimensions=1
  GlobalParams7 : Inport  Port=3  PortDimensions=7
  ApplyMaximumFlow : MinMax  Inputs=2
  BoundRatio : Saturate  UpperLimit=1  LowerLimit=1e-6
  CriticalEnabled : Selector  InputPortWidth=7  IndexOptions=Index vector (dialog)  Indices=7  OutputSizes=1
  CriticalRatio : Fcn  Expr=(2/(u+1))^(u/(u-1))
  EnableForwardFlow : Switch  Criteria=u2 ~= 0
  ForwardFlow : RelationalOperator  Operator=>  OutDataTypeStr=boolean  RndMeth=Simplest
  Gamma : Selector  InputPortWidth=7  IndexOptions=Index vector (dialog)  Indices=4  OutputSizes=1
  GasR : Selector  InputPortWidth=7  IndexOptions=Index vector (dialog)  Indices=5  OutputSizes=1
  IsChoked : RelationalOperator  Operator=<=  OutDataTypeStr=boolean  RndMeth=Simplest
  MassFlowRaw : Product  Inputs=***/
  MuxGammaRatio : Mux  Inputs=2
  PhiChoked : Fcn  Expr=sqrt(u)*(2/(u+1))^((u+1)/(2*(u-1)))
  PhiSubcritical : Fcn  Expr=sqrt(2*u(1)/(u(1)-1)*(u(2)^(2/u(1))-u(2)^((u(1)+1)/u(1))))
  Pin_raw : Selector  InputPortWidth=24  IndexOptions=Index vector (dialog)  Indices=2*UpstreamBoundary  OutputSizes=1
  Pmin : Selector  InputPortWidth=7  IndexOptions=Index vector (dialog)  Indices=2  OutputSizes=1
  PoutPlusMinimumDrop : Sum
  Pout_raw : Selector  InputPortWidth=24  IndexOptions=Index vector (dialog)  Indices=2*DownstreamBoundary  OutputSizes=1
  PressureRatio : Product  Inputs=*/
  ProtectPin : MinMax  Function=max  Inputs=2
  ProtectPout : MinMax  Function=max  Inputs=2
  ProtectTin : MinMax  Function=max  Inputs=2
  RT : Product  Inputs=**
  SelectPhi : Switch  Criteria=u2 ~= 0
  SqrtRT : Math  Operator=sqrt  SignedPower=off  SaturateOnIntegerOverflow=on
  Tin_raw : Selector  InputPortWidth=24  IndexOptions=Index vector (dialog)  Indices=2*UpstreamBoundary-1  OutputSizes=1
  Tmin : Selector  InputPortWidth=7  IndexOptions=Index vector (dialog)  Indices=1  OutputSizes=1
  UseChokedBranch : Logic  AllPortsSameDT=off  OutDataTypeStr=boolean
  Wmax : Selector  InputPortWidth=7  IndexOptions=Index vector (dialog)  Indices=6  OutputSizes=1
  ZeroFlow : Constant  Value=0
  dPmin : Selector  InputPortWidth=7  IndexOptions=Index vector (dialog)  Indices=3  OutputSizes=1
  W_kgps : Outport
  wires:
  ApplyMaximumFlow/1 -> W_kgps/1
  Wmax/1 -> ApplyMaximumFlow/2
  EnableForwardFlow/1 -> ApplyMaximumFlow/1
  ZeroFlow/1 -> EnableForwardFlow/3
  ForwardFlow/1 -> EnableForwardFlow/2
  MassFlowRaw/1 -> EnableForwardFlow/1
  SqrtRT/1 -> MassFlowRaw/4
  EffectiveArea_m2/1 -> MassFlowRaw/3
  SelectPhi/1 -> MassFlowRaw/2
  RT/1 -> SqrtRT/1
  ProtectTin/1 -> RT/2
  GasR/1 -> RT/1
  PhiSubcritical/1 -> SelectPhi/3
  UseChokedBranch/1 -> SelectPhi/2
  PhiChoked/1 -> SelectPhi/1
  CriticalEnabled/1 -> UseChokedBranch/2
  IsChoked/1 -> UseChokedBranch/1
  CriticalRatio/1 -> IsChoked/2
  MuxGammaRatio/1 -> PhiSubcritical/1
  BoundRatio/1 -> IsChoked/1, MuxGammaRatio/2
  Gamma/1 -> MuxGammaRatio/1, PhiChoked/1, CriticalRatio/1
  PressureRatio/1 -> BoundRatio/1
  PoutPlusMinimumDrop/1 -> ForwardFlow/2
  ProtectPin/1 -> MassFlowRaw/1, PressureRatio/2, ForwardFlow/1
  dPmin/1 -> PoutPlusMinimumDrop/2
  ProtectPout/1 -> PressureRatio/1, PoutPlusMinimumDrop/1
  Pout_raw/1 -> ProtectPout/1
  Pmin/1 -> ProtectPout/2, ProtectPin/2
  Pin_raw/1 -> ProtectPin/1
  Tmin/1 -> ProtectTin/2
  Tin_raw/1 -> ProtectTin/1
  GlobalParams7/1 -> CriticalEnabled/1, Wmax/1, GasR/1, Gamma/1, dPmin/1, Pmin/1, Tmin/1
  BoundaryTP24/1 -> Pout_raw/1, Pin_raw/1, Tin_raw/1

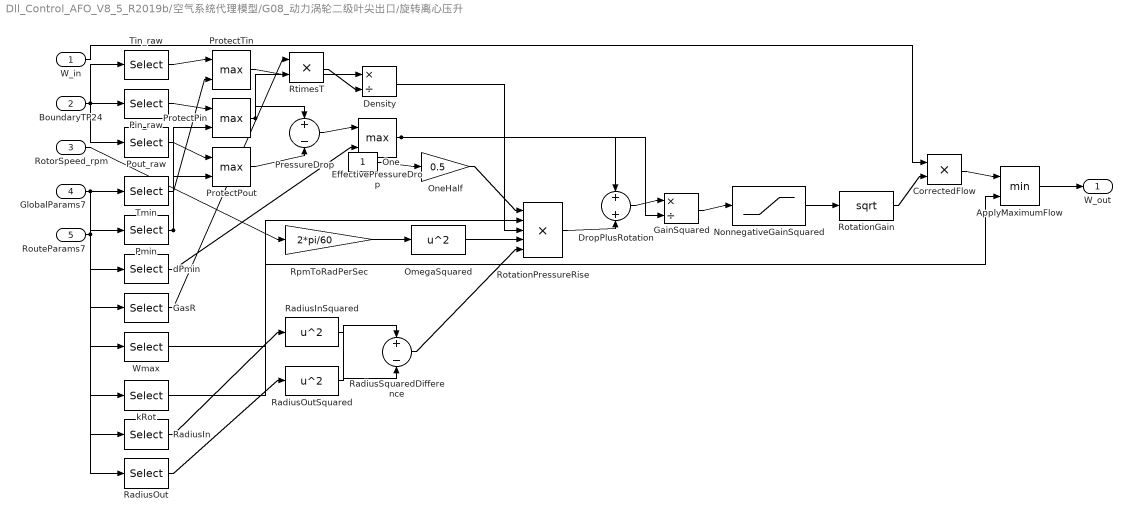
== system Dll_Control_AFO_V8_5_R2019b/空气系统代理模型/G08_动力涡轮二级叶尖出口/旋转离心压升 ==
  W_in : Inport  PortDimensions=1
  BoundaryTP24 : Inport  Port=2  PortDimensions=24
  RotorSpeed_rpm : Inport  Port=3  PortDimensions=1
  GlobalParams7 : Inport  Port=4  PortDimensions=7
  RouteParams7 : Inport  Port=5  PortDimensions=7
  ApplyMaximumFlow : MinMax  Inputs=2
  CorrectedFlow : Product  Inputs=**
  Density : Product  Inputs=*/
  DropPlusRotation : Sum
  EffectivePressureDrop : MinMax  Function=max  Inputs=2
  GainSquared : Product  Inputs=*/
  GasR : Selector  InputPortWidth=7  IndexOptions=Index vector (dialog)  Indices=5  OutputSizes=1
  NonnegativeGainSquared : Saturate  UpperLimit=16  LowerLimit=0
  OmegaSquared : Math  Operator=square  SignedPower=off  SaturateOnIntegerOverflow=on
  One : Constant
  OneHalf : Gain  Gain=0.5
  Pin_raw : Selector  InputPortWidth=24  IndexOptions=Index vector (dialog)  Indices=2*UpstreamBoundary  OutputSizes=1
  Pmin : Selector  InputPortWidth=7  IndexOptions=Index vector (dialog)  Indices=2  OutputSizes=1
  Pout_raw : Selector  InputPortWidth=24  IndexOptions=Index vector (dialog)  Indices=2*DownstreamBoundary  OutputSizes=1
  PressureDrop : Sum  Inputs=+-
  ProtectPin : MinMax  Function=max  Inputs=2
  ProtectPout : MinMax  Function=max  Inputs=2
  ProtectTin : MinMax  Function=max  Inputs=2
  RadiusIn : Selector  InputPortWidth=7  IndexOptions=Index vector (dialog)  Indices=3  OutputSizes=1
  RadiusInSquared : Math  Operator=square  SignedPower=off  SaturateOnIntegerOverflow=on
  RadiusOut : Selector  InputPortWidth=7  IndexOptions=Index vector (dialog)  Indices=4  OutputSizes=1
  RadiusOutSquared : Math  Operator=square  SignedPower=off  SaturateOnIntegerOverflow=on
  RadiusSquaredDifference : Sum  Inputs=+-
  RotationGain : Math  Operator=sqrt  SignedPower=off  SaturateOnIntegerOverflow=on
  RotationPressureRise : Product  Inputs=*****
  RpmToRadPerSec : Gain  Gain=2*pi/60
  RtimesT : Product  Inputs=**
  Tin_raw : Selector  InputPortWidth=24  IndexOptions=Index vector (dialog)  Indices=2*UpstreamBoundary-1  OutputSizes=1
  Tmin : Selector  InputPortWidth=7  IndexOptions=Index vector (dialog)  Indices=1  OutputSizes=1
  Wmax : Selector  InputPortWidth=7  IndexOptions=Index vector (dialog)  Indices=6  OutputSizes=1
  dPmin : Selector  InputPortWidth=7  IndexOptions=Index vector (dialog)  Indices=3  OutputSizes=1
  kRot : Selector  InputPortWidth=7  IndexOptions=Index vector (dialog)  Indices=2  OutputSizes=1
  W_out : Outport
  wires:
  ApplyMaximumFlow/1 -> W_out/1
  Wmax/1 -> ApplyMaximumFlow/2
  CorrectedFlow/1 -> ApplyMaximumFlow/1
  RotationGain/1 -> CorrectedFlow/2
  W_in/1 -> CorrectedFlow/1
  NonnegativeGainSquared/1 -> RotationGain/1
  GainSquared/1 -> NonnegativeGainSquared/1
  DropPlusRotation/1 -> GainSquared/1
  RotationPressureRise/1 -> DropPlusRotation/2
  EffectivePressureDrop/1 -> GainSquared/2, DropPlusRotation/1
  dPmin/1 -> EffectivePressureDrop/2
  PressureDrop/1 -> EffectivePressureDrop/1
  ProtectPout/1 -> PressureDrop/2
  RadiusSquaredDifference/1 -> RotationPressureRise/5
  OmegaSquared/1 -> RotationPressureRise/4
  Density/1 -> RotationPressureRise/3
  kRot/1 -> RotationPressureRise/2
  OneHalf/1 -> RotationPressureRise/1
  One/1 -> OneHalf/1
  RadiusInSquared/1 -> RadiusSquaredDifference/2
  RadiusOutSquared/1 -> RadiusSquaredDifference/1
  RadiusOut/1 -> RadiusOutSquared/1
  RadiusIn/1 -> RadiusInSquared/1
  RpmToRadPerSec/1 -> OmegaSquared/1
  RotorSpeed_rpm/1 -> RpmToRadPerSec/1
  RtimesT/1 -> Density/2
  ProtectPin/1 -> PressureDrop/1, Density/1
  ProtectTin/1 -> RtimesT/2
  GasR/1 -> RtimesT/1
  Pout_raw/1 -> ProtectPout/1
  Pmin/1 -> ProtectPout/2, ProtectPin/2
  Pin_raw/1 -> ProtectPin/1
  Tmin/1 -> ProtectTin/2
  Tin_raw/1 -> ProtectTin/1
  RouteParams7/1 -> RadiusOut/1, RadiusIn/1, kRot/1
  GlobalParams7/1 -> Wmax/1, GasR/1, dPmin/1, Pmin/1, Tmin/1
  BoundaryTP24/1 -> Pout_raw/1, Pin_raw/1, Tin_raw/1

== system Dll_Control_AFO_V8_5_R2019b/空气系统代理模型/G08_动力涡轮二级叶尖出口/流路可调参数 ==
  Mux_RouteParams7 : Mux  Inputs=7
  kRot : Constant  Value=0.5
  内半径_m : Constant  Value=0.076999999999999999
  初值流量_kgps : Constant  Value=0.030201306673577899
  外半径_m : Constant  Value=0.078
  时间常数_s : Constant  Value=0
  等效面积缩放 : Constant  Value=1.0010962365271501
  篦齿修正系数 : Constant
  RouteParams7 : Outport
  wires:
  等效面积缩放/1 -> Mux_RouteParams7/1
  kRot/1 -> Mux_RouteParams7/2
  内半径_m/1 -> Mux_RouteParams7/3
  外半径_m/1 -> Mux_RouteParams7/4
  时间常数_s/1 -> Mux_RouteParams7/5
  初值流量_kgps/1 -> Mux_RouteParams7/6
  篦齿修正系数/1 -> Mux_RouteParams7/7
  Mux_RouteParams7/1 -> RouteParams7/1

== system Dll_Control_AFO_V8_5_R2019b/空气系统代理模型/G08_动力涡轮二级叶尖出口/盘腔热动态 ==
  W_in : Inport  PortDimensions=1
  RouteParams7 : Inport  Port=2  PortDimensions=7
  Alpha : Fcn  Expr=exp(-SampleTime_s/u)
  DynamicOrBypass : Switch  Criteria=u2 ~= 0
  One : Constant
  OneMinusAlpha : Sum  Inputs=+-
  ProtectTau : Saturate  UpperLimit=inf  LowerLimit=1e-9
  State : UnitDelay  InitialCondition=InitialFlowValue  SampleTime=SampleTime_s  HasFrameUpgradeWarning=on
  Tau_s : Selector  InputPortWidth=7  IndexOptions=Index vector (dialog)  Indices=5  OutputSizes=1
  Update : Sum
  UseBypass : simulink/Logic and Bit Operations/Compare To Constant  relop=<=  const=1e-12  OutDataTypeStr=boolean
  WeightedInput : Product  Inputs=**
  WeightedState : Product  Inputs=**
  W_out : Outport
  wires:
  DynamicOrBypass/1 -> W_out/1
  UseBypass/1 -> DynamicOrBypass/2
  Update/1 -> DynamicOrBypass/3, State/1
  WeightedState/1 -> Update/2
  WeightedInput/1 -> Update/1
  State/1 -> WeightedState/1
  OneMinusAlpha/1 -> WeightedInput/2
  W_in/1 -> DynamicOrBypass/1, WeightedInput/1
  Alpha/1 -> WeightedState/2, OneMinusAlpha/2
  One/1 -> OneMinusAlpha/1
  ProtectTau/1 -> Alpha/1
  Tau_s/1 -> UseBypass/1, ProtectTau/1
  RouteParams7/1 -> Tau_s/1

== system Dll_Control_AFO_V8_5_R2019b/空气系统代理模型/G08_动力涡轮二级叶尖出口/辨识等效面积 ==
  BoundaryTP24 : Inport  PortDimensions=24
  IdentifiedAreaLaw : MATLAB Function  TreatAsAtomicUnit=on
  EffectiveArea_m2 : Outport
  wires:
  BoundaryTP24/1 -> IdentifiedAreaLaw/1(boundaryTP24)
  IdentifiedAreaLaw/1(area) -> EffectiveArea_m2/1

== system Dll_Control_AFO_V8_5_R2019b/滑油系统代理模型/滑油系统代理核心/支路_流量压力分配/核心流量压力计算 ==
  u26 : Inport
  FCN_FP_Formula : MATLAB Function  TreatAsAtomicUnit=on
  FCN_FP_Predict : MATLAB Function  TreatAsAtomicUnit=on
  状态拆分 : Demux  Outputs=7
  输出融合 : Sum
  QA_m3_s : Outport
  QB_m3_s : Outport  Port=2
  PA_Pa : Outport  Port=3
  PB_Pa : Outport  Port=4
  QG_m3_s : Outport  Port=5
  Pman_Pa : Outport  Port=6
  Pret_Pa : Outport  Port=7
  wires:
  u26/1 -> FCN_FP_Predict/1(u), FCN_FP_Formula/1(u)
  FCN_FP_Predict/1(y) -> 输出融合/1
  FCN_FP_Formula/1(y) -> 输出融合/2
  输出融合/1 -> 状态拆分/1
  状态拆分/1 -> QA_m3_s/1  "QA_m3_s"
  状态拆分/2 -> QB_m3_s/1  "QB_m3_s"
  状态拆分/3 -> PA_Pa/1  "PA_Pa"
  状态拆分/4 -> PB_Pa/1  "PB_Pa"
  状态拆分/5 -> QG_m3_s/1  "QG_m3_s"
  状态拆分/6 -> Pman_Pa/1  "Pman_Pa"
  状态拆分/7 -> Pret_Pa/1  "Pret_Pa"

== matlab function Dll_Control_AFO_V8_5_R2019b/Turboshaft Engine Control System/MATLAB Function1 ==
  data: err_Mkp input; MkpMax input; Mkp input; y output; Ts input
function y = fcn(err_Mkp, MkpMax, Mkp, Ts)

% if MkpMax < Mkp
%     y = err_Mkp*4*Ts;
% else
%     y = 1e3;
% end
K = interp1([0 5 10   20 50 100   1000], [4  4  8   12  16  20    24], abs(err_Mkp), 'linear', 'extrap');
% K = 4;
    y = err_Mkp*K*Ts;

== matlab function Dll_Control_AFO_V8_5_R2019b/Turboshaft Engine Control System/MATLAB Function ==
  data: err_T45 input; T45Max input; T45 input; y output; Ts input
function y = fcn(err_T45, T45Max, T45, Ts)

% if T45Max < T45
%     y = err_T45*4*Ts;
% else
%     y = 1e3;
% end
K = interp1([0 5 10   20 50 100   1000], [4  4  8   12  16  20    24], abs(err_T45), 'linear', 'extrap');

    y = err_T45*K*Ts;

== matlab function Dll_Control_AFO_V8_5_R2019b/空气系统代理模型/G01_燃气涡轮一级进口/辨识等效面积/IdentifiedAreaLaw ==
  data: boundaryTP24 input; area output
function area = f(boundaryTP24)
%#codegen
indices = [1 2 3 4 5 6 7 8 17 18 19 20 23 24];
center = [1143.9851310850022 107995.87488112479 1622.2348189112549 1499845.6209487044 1622.2348189112549 1499845.6209487044 1622.2348189112549 1499845.6209487044 1383.1099749981283 803920.74791491474 701.05126049106082 1554244.1667862225 701.05126049106082 1554244.1667862225];
scale = [95.954376618145574 621.80388296676324 138.0910860203727 100531.17106538037 138.0910860203727 100531.17106538037 138.0910860203727 100531.17106538037 117.02019532436552 50576.000521072063 15.06449605558042 104177.37934236297 15.06449605558042 104177.37934236297];
beta = [-8.286477915750444 0.15372495212206674 0.02711540262909282 -0.074075861371024773 -0.0042825662002896883 -0.074075861358680467 -0.0042825662002638791 -0.074075861358680467 -0.0042825661928602822 0.019318741308003748 -0.0040896044626861491 0.0043674149989198123 -0.0042825752201098004 0.0043674150179875198 -0.0042825692753761741];
features = zeros(1, 14);
for k = 1:14
    features(k) = (boundaryTP24(indices(k)) - center(k)) / scale(k);
end
logArea = beta(1);
for k = 1:14
    logArea = logArea + features(k) * beta(k + 1);
end
logArea = min(0, max(-30, logArea));
area = exp(logArea);
end
